simulink library "Linkage_DW_Pullrod_NoSteer"  (R2025a)
settings: Solver=VariableStepAuto  StartTime=0.0  StopTime=10.0  RelTol=1e-3
undefined symbols (not defined in the file): Ac, Af, Ar, InitLinkage, Left, Linkage, Visual, X, Y, Z
libraries: sm_lib x25, Linkage_Arms x5, Suspension_Utilities x4, Linkage_Shock x1, Linkage_Uprights x1
(part 1 of 2)
Description:
  | Component of Simscape Vehicle Templates Library
  | 
  | Copyright 2018-2026 The MathWorks, Inc.
settings Model: Creator=smiller  LastModifiedBy=smiller
settings SolverCC: AlgebraicLoopSolver=TrustRegion
settings DataIOCC: ReturnWorkspaceOutputs=off
settings OptimizationCC: ReuseModelBlockBuffer=off
settings DebuggingCC: UnconnectedInputMsg=warning  UnconnectedOutputMsg=warning  UnconnectedLineMsg=warning  ArithmeticOperatorsInVariantConditions=warning
settings ModelReferenceCC: EnableRefExpFcnMdlSchedulingChecks=on
settings SFSimCC: CustomCodeUndefinedFunction=UseInterfaceOnly
settings RTWCC: GPUComputeCapability=3.5

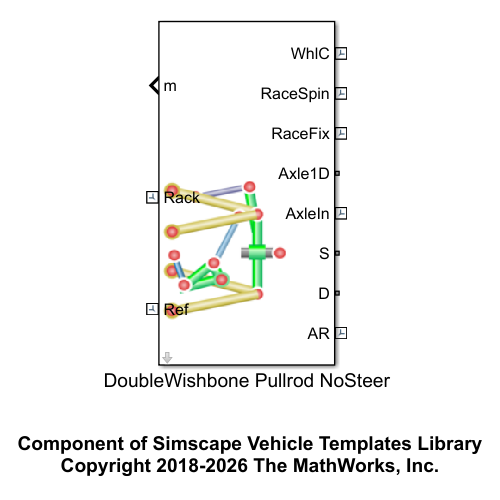
[thumbnail: Simulink's stored preview of the top-level diagram]
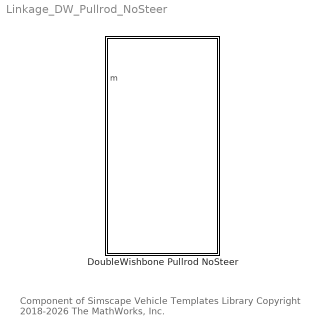
== system Linkage_DW_Pullrod_NoSteer ==
  note: Component of Simscape Vehicle Templates Library
      | Copyright 2018-2026 The MathWorks, Inc.
  DoubleWishbone Pullrod NoSteer : Subsystem  VariantControl=DoubleWishbonePullrodNoSteer  mask(Double-Wishbone Suspension, Pullrod, no Steer){popup_leftRight=Left, hp_in_f_ua=Linkage.UpperWishbone.sInboardF.Value, hp_in_r_ua=Linkage.UpperWishbone.sInboardR.Value, hp_out_ua=Linkage.UpperWishbone.sOutboard.Value, hp_in_f_la=Linkage.LowerWishbone.sInboardF.Value, hp_in_r_la=Linkage.LowerWishbone.sInboardR.Value, hp_out_la=Linkage.LowerWishbone.sOutboard.Value, hp_pullrod_out=Linkage.Pullrod.sUpperArm.Value, hp_pullrod_in=Linkage.Pullrod.sBellcrank.Value, hp_bcr_pivot=Linkage.Bellcrank.sPivot.Value, hp_arb=Linkage.Bellcrank.sAntiRollBar.Value, hp_upr_cg=Linkage.Upright.sCG.Value, hp_upr_wc=Linkage.Upright.sWheelCentre.Value, hp_upr_rod=Linkage.TrackRod.sOutboard.Value, hp_uar_rod=Linkage.TrackRod.sInboard.Value, hp_spr_body=Linkage.Shock.sTop.Value, hp_spr_bcr=Linkage.Shock.sBottom.Value, clr_hp=Visual.hp.clr, opc_hp=Visual.hp.opc, size_hp=Visual.hp.rad, Upper_Arm_to_Subframe=Linkage.Upper_Arm_to_Subframe, ua_mass=Linkage.UpperWishbone.m.Value, clr_ua=Visual.UpperArm.clr, opc_ua=Visual.part.opc, radius_ua=Visual.UpperArm.rad, Lower_Arm_to_Subframe=Linkage.Lower_Arm_to_Subframe, la_mass=Linkage.LowerWishbone.m.Value, clr_la=Visual.LowerArm.clr, opc_la=Visual.part.opc, radius_la=Visual.LowerArm.rad, shock_pist_mass=Linkage.Shock.mPiston.Value, shock_cyl_mass=Linkage.Shock.mCylinder.Value, up_lim_bumpstop=Linkage.Endstop.xMax.Value, low_lim_bumpstop=Linkage.Endstop.xMin.Value, clr_conn_shock=Visual.hp.clr, opc_conn_shock=Visual.hp.opc, size_conn_shock=Visual.hp.rad, clr_shock_cyl=Visual.Shock.cyl.clr, opc_shock_cyl=Visual.part.opc, radius_shock_cyl=Visual.Shock.cyl.rad, clr_shock_piston=Visual.Shock.piston.clr, opc_shock_piston=Visual.part.opc, clr_shock_bumpstop=Visual.Shock.bumpstop.clr, opc_shock_bumpstop=Visual.part.opc, deadvol_len_shock_cyl=Visual.Shock.dead_length, piston_len_shock=Visual.Shock.piston.len, cyl_cap_len_shock=Visual.Shock.cap.len, bumpstop_len_shock=Visual.Shock.bumpstop.len, upr_mass=Linkage.Upright.m.Value, atoe=Linkage.Upright.aToe.Value, acamber=Linkage.Upright.aCamber.Value, axle_len=Linkage.Upright.xAxle.Value, axle_whlc_to_bearing=Linkage.Upright.xWCtoBearing.Value, axle_mass=Linkage.Upright.mAxle.Value, clr_conn_upr=Visual.hp.clr, opc_conn_upr=Visual.hp.opc, size_conn_upr=Visual.hp.rad, clr_upr=Visual.Upright.clr, opc_upr=Visual.part.opc, radius_upr=Visual.Upright.rad, clr_axle=Visual.Axle.clr, opc_axle=Visual.part.opc, radius_axle=Visual.Axle.rad, rod_mass=Linkage.TrackRod.m.Value, clr_conn_rod=Visual.hp.clr, opc_conn_rod=Visual.hp.opc, size_conn_rod=Visual.hp.rad, clr_rod=Visual.TrackRod.clr, opc_rod=Visual.part.opc, radius_rod=Visual.TrackRod.rad, bcr_mass=Linkage.Bellcrank.m.Value, clr_bcr=Visual.Bellcrank.clr, opc_bcr=Visual.part.opc, radius_bcr=Visual.Bellcrank.rad, pullrod_mass=Linkage.Pullrod.m.Value, clr_conn_pullrod=Visual.hp.clr, opc_conn_pullrod=Visual.hp.opc, size_conn_pullrod=Visual.hp.rad, clr_pullrod=Visual.Pullrod.clr, opc_pullrod=Visual.part.opc, radius_pullrod=Visual.Pullrod.rad, whl_init_spd_lr=InitLinkage.nWheel.Value}
      mask prompts: popup_leftRight "Left/Right"; hp_in_f_ua "Upper Arm Front [xyz] (m)"; hp_in_r_ua "Upper Arm Rear [xyz] (m)"; hp_out_ua "Upper Arm Outboard [xyz] (m)"; hp_in_f_la "Lower Arm Front [xyz] (m)"; hp_in_r_la "Lower Arm Rear [xyz] (m)"; hp_out_la "Lower Arm Outboard [xyz] (m)"; hp_pullrod_out "Pullrod Upper Arm [xyz] (m)"; hp_pullrod_in "Pullrod Bellcrank [xyz] (m)"; hp_bcr_pivot "Bellcrank Pivot [xyz] (m)"; hp_arb "HP Bellcrank ARB [xyz] (m)"; hp_upr_cg "Upright CG [xyz] (m)"; hp_upr_wc "Wheel Center [xyz] (m)"; hp_upr_rod "Track Rod Outboard [xyz] (m)"; hp_uar_rod "Track Rod Inboard [xyz] (m)"; hp_spr_body "Spring Body [xyz] (m)"; hp_spr_bcr "Spring Bellcrank [xyz] (m)"; Upper_Arm_to_Subframe "Subframe Connection"; ua_mass "Mass (kg)"; clr_ua "Color [RGB]"; opc_ua "Opacity (0-1)"; radius_ua "Radius (m)"; Lower_Arm_to_Subframe "Subframe Connection"; la_mass "Mass (kg)"; clr_la "Color [RGB]"; opc_la "Opacity (0-1)"; radius_la "Radius (m)"; shock_pist_mass "Piston Mass (kg)"; shock_cyl_mass "Cylinder Mass (kg)"; up_lim_bumpstop "Upper Limit (m)"; low_lim_bumpstop "Lower Limit (m)"; deadvol_len_shock_cyl "Dead Volume Height (m)"; piston_len_shock "Piston Length (m)"; cyl_cap_len_shock "Cylinder Cap Length (m)"; bumpstop_len_shock "Bumpstop Length (m)"; upr_mass "Mass (kg)"; atoe "Toe Angle (deg)"; acamber "Camber Angle (deg)"; axle_len "Axle Length (m)"; axle_whlc_to_bearing "Distance Wheel Ctr to Bearing (m)"; axle_mass "Axle Mass (kg)"; rod_mass "Mass (kg)"; bcr_mass "Mass (kg)"; pullrod_mass "Mass (kg)"; whl_init_spd_lr "Initial Wheel Speed (rad/s)"
      mask help: This models a non-steerable double-wishbone suspension with a rod connecting the upper arm and a bellcrank.
      mask init:
      | if(popup_leftRight == 1)
      |     rhs_susp = 1;
      |     %whlind = 1;
      |     whl_init_spd = whl_init_spd_lr(1);
      | elseif(popup_leftRight == 2)
      |     rhs_susp = -1;
      |     %whlind = 2;
      |     whl_init_spd = whl_init_spd_lr(2);
      | end
      mask Help: web('sm_car_doc_susp_double_wishbone.html')
      mask TypeOptions popup_leftRight:
      | Bellcrank/popup_leftRight | HP Bellcrank/popup_leftRight | HP LA/popup_leftRight | HP UA/popup_leftRight | Hardpoints/popup_leftRight | Lower Arm/popup_leftRight | Pull
      | Rod/popup_leftRight | Track Rod/popup_leftRight | Upper Arm/popup_leftRight | Upright/popup_leftRight
      mask TypeOptions hp_in_f_ua: HP UA/hp_f | Hardpoints/hp_in_f_ua | Upper Arm/hp_in_f
      mask TypeOptions hp_in_r_ua: HP UA/hp_r | Hardpoints/hp_in_r_ua | Upper Arm/hp_in_r
      mask TypeOptions hp_out_ua: Upper Arm/hp_out | Upright/hp_ua_out
      mask TypeOptions hp_in_f_la: HP LA/hp_f | Hardpoints/hp_in_f_la | Lower Arm/hp_in_f
      mask TypeOptions hp_in_r_la: HP LA/hp_r | Hardpoints/hp_in_r_la | Lower Arm/hp_in_r
      mask TypeOptions hp_out_la: Lower Arm/hp_out | Upright/hp_la_out
      mask TypeOptions hp_pullrod_out:
      | Pull
      | Rod/hp_out | Upper Arm/hp_rod
      mask TypeOptions hp_pullrod_in:
      | Bellcrank/hp_rod | HP Bellcrank/hp_2 | Pull
      | Rod/hp_in
      mask TypeOptions hp_bcr_pivot: Bellcrank/hp_bcr_pivot | HP Bellcrank/hp_1 | Hardpoints/hp_bellcrank
      mask TypeOptions hp_arb: Bellcrank/hp_arb
      mask TypeOptions hp_upr_cg: Upright/hp_upr_cg
      mask TypeOptions hp_upr_wc: Upright/hp_upr_wc
      mask TypeOptions hp_upr_rod: Track Rod/hp_out | Upright/hp_upr_rod
      mask TypeOptions hp_uar_rod: Upper Arm/hp_r_upr | Track Rod/hp_in
      mask TypeOptions hp_spr_body: Hardpoints/hp_spr_top | Shock/hp_spr_top
      mask TypeOptions hp_spr_bcr: Bellcrank/hp_bcr_shock | HP Bellcrank/hp_3 | Shock/hp_spr_bot
      mask TypeOptions clr_hp: Hardpoints/clr_hp
      mask TypeOptions opc_hp: Hardpoints/opc_hp
      mask TypeOptions size_hp: Hardpoints/size_hp
      mask TypeOptions ua_mass: Upper Arm/ua_mass
      mask TypeOptions clr_ua: Upper Arm/clr_ua
      mask TypeOptions opc_ua: Upper Arm/opc_ua
      mask TypeOptions radius_ua: Upper Arm/radius_ua
      mask TypeOptions la_mass: Lower Arm/arm_mass
      mask TypeOptions clr_la: Lower Arm/clr_arm
      mask TypeOptions opc_la: Lower Arm/opc_arm
      mask TypeOptions radius_la: Lower Arm/radius_arm
      mask TypeOptions shock_pist_mass: Shock/shock_pist_mass
      mask TypeOptions shock_cyl_mass: Shock/shock_cyl_mass
      mask TypeOptions up_lim_bumpstop: Shock/up_lim_bumpstop
      mask TypeOptions low_lim_bumpstop: Shock/low_lim_bumpstop
      mask TypeOptions clr_conn_shock: Shock/clr_conn_shock
      mask TypeOptions opc_conn_shock: Shock/opc_conn_shock
      mask TypeOptions size_conn_shock: Shock/size_conn_shock
      mask TypeOptions clr_shock_cyl: Shock/clr_shock_cyl
      mask TypeOptions opc_shock_cyl: Shock/opc_shock_cyl
      mask TypeOptions radius_shock_cyl: Shock/radius_shock_cyl
      mask TypeOptions clr_shock_piston: Shock/clr_shock_piston
      mask TypeOptions opc_shock_piston: Shock/opc_shock_piston
      mask TypeOptions clr_shock_bumpstop: Shock/clr_shock_bumpstop
      mask TypeOptions opc_shock_bumpstop: Shock/opc_shock_bumpstop
      mask TypeOptions deadvol_len_shock_cyl: Shock/deadvol_len_shock_cyl
      mask TypeOptions piston_len_shock: Shock/piston_len_shock
      mask TypeOptions cyl_cap_len_shock: Shock/cyl_cap_len_shock
      mask TypeOptions bumpstop_len_shock: Shock/bumpstop_len_shock
      mask TypeOptions upr_mass: Upright/upr_mass
      mask TypeOptions atoe: Upright/atoe
      mask TypeOptions acamber: Upright/acamber
      mask TypeOptions axle_len: Upright/axle_len
      mask TypeOptions axle_whlc_to_bearing: Upright/axle_whlc_to_bearing
      mask TypeOptions axle_mass: Upright/axle_mass
      mask TypeOptions clr_conn_upr: Upright/clr_conn_upr
      mask TypeOptions opc_conn_upr: Upright/opc_conn_upr
      mask TypeOptions size_conn_upr: Upright/size_conn_upr
      mask TypeOptions clr_upr: Upright/clr_upr
      mask TypeOptions opc_upr: Upright/opc_upr
      mask TypeOptions radius_upr: Upright/radius_upr
      mask TypeOptions clr_axle: Upright/clr_axle
      mask TypeOptions opc_axle: Upright/opc_axle
      mask TypeOptions radius_axle: Upright/radius_axle
      mask TypeOptions rod_mass: Track Rod/rod_mass
      mask TypeOptions clr_conn_rod: Track Rod/clr_conn_rod
      mask TypeOptions opc_conn_rod: Track Rod/opc_conn_rod
      mask TypeOptions size_conn_rod: Track Rod/size_conn_rod
      mask TypeOptions clr_rod: Track Rod/clr_rod
      mask TypeOptions opc_rod: Track Rod/opc_rod
      mask TypeOptions radius_rod: Track Rod/radius_rod
      mask TypeOptions bcr_mass: Bellcrank/bcr_mass
      mask TypeOptions clr_bcr: Bellcrank/clr_bcr
      mask TypeOptions opc_bcr: Bellcrank/opc_bcr
      mask TypeOptions radius_bcr: Bellcrank/radius_bcr
      mask TypeOptions pullrod_mass:
      | Pull
      | Rod/rod_mass
      mask TypeOptions clr_conn_pullrod:
      | Pull
      | Rod/clr_conn_rod
      mask TypeOptions opc_conn_pullrod:
      | Pull
      | Rod/opc_conn_rod
      mask TypeOptions size_conn_pullrod:
      | Pull
      | Rod/size_conn_rod
      mask TypeOptions clr_pullrod:
      | Pull
      | Rod/clr_rod
      mask TypeOptions opc_pullrod:
      | Pull
      | Rod/opc_rod
      mask TypeOptions radius_pullrod:
      | Pull
      | Rod/radius_rod
      mask DialogControl cont_hp Prompt: Hardpoints
      mask DialogControl cont_vis_hp Prompt: Visualization
      mask DialogControl text_clr_hp Prompt: Color [RGB]
      mask DialogControl text_opc_hp Prompt: Opac. (0-1)
      mask DialogControl text_size_hp Prompt: Size (m)
      mask DialogControl text_hp Prompt: Hardpoints
      mask DialogControl cont_ua Prompt: UA
      mask DialogControl cont_vis_ua Prompt: Visualization
      mask DialogControl cont_la Prompt: LA
      mask DialogControl cont_vis_la Prompt: Visualization
      mask DialogControl cont_shock Prompt: Shock
      mask DialogControl cont_parts Prompt: Parts
      mask DialogControl cont_bumpstop Prompt: Bumpstop
      mask DialogControl cont_vis_shock Prompt: Visualization
      mask DialogControl text_clr_shock Prompt: Color  [RGB]
      mask DialogControl text_opc_shock Prompt: Opac. (0-1)
      mask DialogControl text_size_shock Prompt: Size (m)
      mask DialogControl text_conn_shock Prompt: Connections
      mask DialogControl text_shock_shock Prompt: Cylinder
      mask DialogControl text_shock_piston Prompt: Piston
      mask DialogControl text_piston_radius Prompt: <cylinder radius>
      mask DialogControl text_shock_bumpstop Prompt: Bumpstop
      mask DialogControl text_bumpstop_radius Prompt: <cylinder radius>
      mask DialogControl cont_upright Prompt: Upright
      mask DialogControl grp_upright Prompt: Upright
      mask DialogControl grp_upright_axle Prompt: Axle
      mask DialogControl cont_vis_upr Prompt: Visualization
      mask DialogControl text_clr_upr Prompt: Color [RGB]
      mask DialogControl text_opc_upr Prompt: Opac. (0-1)
      mask DialogControl text_size_upr Prompt: Size (m)
      mask DialogControl text_conn_upr Prompt: Connections
      mask DialogControl text_upright Prompt: Upright
      mask DialogControl text_axle Prompt: Axle
      mask DialogControl cont_steer Prompt: Steer
      mask DialogControl grp_rod Prompt: Rod
      mask DialogControl cont_vis_rod Prompt: Visualization
      mask DialogControl text_clr_rod Prompt: Color [RGB]
      mask DialogControl text_opc_rod Prompt: Opac. (0-1)
      mask DialogControl text_size_rod Prompt: Size (m)
      mask DialogControl text_conn_rod Prompt: Connections
      mask DialogControl text_rod_rod Prompt: Rod
      mask DialogControl Container23 Prompt: Bellcrank
      mask DialogControl grp_bellcrank Prompt: Bellcrank
      mask DialogControl cont_vis_bellcrank Prompt: Visualization
      mask DialogControl text_clr_bellcrank Prompt: Color [RGB]
      mask DialogControl text_opc_bellcrank Prompt: Opac. (0-1)
      mask DialogControl text_size_bellcrank Prompt: Size (m)
      mask DialogControl text_bellcrank Prompt: Bellcrank
      mask DialogControl cont_pull Prompt: Pullrod
      mask DialogControl grp_pullrod Prompt: Pullrod
      mask DialogControl cont_vis_pullrod Prompt: Visualization
      mask DialogControl text_clr_pullrod Prompt: Color [RGB]
      mask DialogControl text_opc_pullrod Prompt: Opac. (0-1)
      mask DialogControl text_size_pullrod Prompt: Size (m)
      mask DialogControl text_conn_pullrod Prompt: Connections
      mask DialogControl text_pullrod Prompt: Pullrod
      mask DialogControl cont_init Prompt: Initial
      mask Display: image('sm_car_vehicle_linkage_dw_pullrod_noSteer_IMAGE.png');

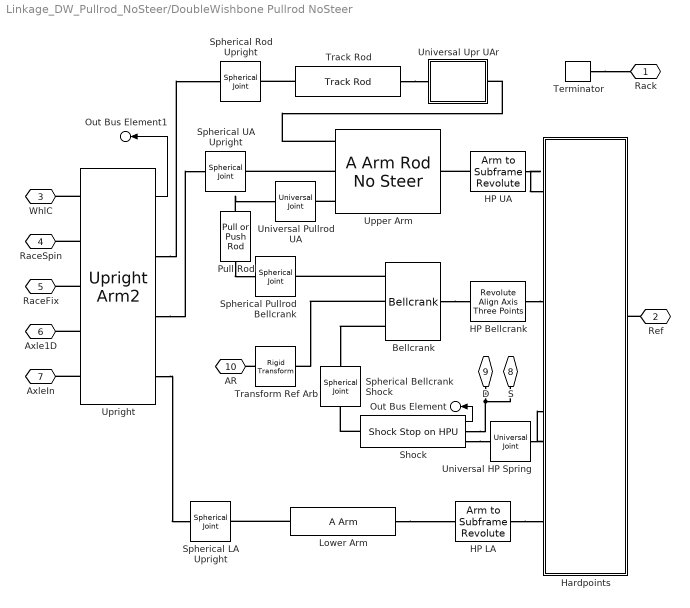
== system Linkage_DW_Pullrod_NoSteer/DoubleWishbone Pullrod NoSteer ==
  Bellcrank : Linkage_Arms/Bellcrank  popup_leftRight=Left  hp_bcr_pivot=hp_bcr_pivot  hp_bcr_shock=hp_spr_bcr  hp_rod=hp_pullrod_in  hp_arb=hp_arb  bcr_mass=bcr_mass  clr_bcr=clr_bcr  opc_bcr=opc_bcr  radius_bcr=radius_bcr
  HP Bellcrank : Suspension_Utilities/Revolute Align Axis Three Points  popup_leftRight=Left  hp_1=hp_bcr_pivot  hp_2=hp_pullrod_in  hp_3=hp_spr_bcr  positionTargetSpecify=on  PositionTargetValue=0
  HP LA : Suspension_Utilities/Arm to Subframe Revolute  VariantControl=Variant1  LabelModeActiveChoice=Rigid_1Rev  popup_leftRight=Left  hp_f=hp_in_f_la  hp_r=hp_in_r_la  Connection=Lower_Arm_to_Subframe  VariantLabel=Lower_Arm_to_Subframe.class.Value
      settings: AttributesFormatString=%<ActiveVariant>
  HP UA : Suspension_Utilities/Arm to Subframe Revolute  VariantControl=Variant1  LabelModeActiveChoice=Rigid_1Rev  popup_leftRight=Left  hp_f=hp_in_f_ua  hp_r=hp_in_r_ua  Connection=Upper_Arm_to_Subframe  VariantLabel=Upper_Arm_to_Subframe.class.Value
      settings: AttributesFormatString=%<ActiveVariant>
  Hardpoints : Subsystem  mask{popup_leftRight=Left, hp_in_f_ua=hp_in_f_ua, hp_in_r_ua=hp_in_r_ua, hp_in_f_la=hp_in_f_la, hp_in_r_la=hp_in_r_la, hp_bellcrank=hp_bcr_pivot, hp_spr_top=hp_spr_body, clr_hp=clr_hp, opc_hp=opc_hp, size_hp=size_hp}
      mask prompts: popup_leftRight "Left/Right"; hp_in_f_ua "Upper Arm Front [xyz] (m)"; hp_in_r_ua "Upper Arm Rear [xyz] (m)"; hp_in_f_la "Lower Arm Front [xyz] (m)"; hp_in_r_la "Lower Arm Rear [xyz] (m)"; hp_bellcrank "Bellcrank Pivot [xyz] (m)"; hp_spr_top "Spring [xyz] (m)"
      mask init:
      | % Set parameter for mirroring (+y or -y)
      | if(popup_leftRight == 1)
      |     rhs_susp = 1;    
      | elseif(popup_leftRight == 2)
      |     rhs_susp = -1;
      | end
      | 
      | rhs_hp = [1 rhs_susp 1];
      mask TypeOptions popup_leftRight: Left | Right
      mask TypeOptions clr_hp: Subsystem/Vis HP LAf/GraphicDiffuseColor | Vis HP LAr/GraphicDiffuseColor | Vis HP Spring/GraphicDiffuseColor | Vis HP UAf/GraphicDiffuseColor | Vis HP UAr/GraphicDiffuseColor
      mask TypeOptions opc_hp: Subsystem/Vis HP LAf/GraphicOpacity | Vis HP LAr/GraphicOpacity | Vis HP Spring/GraphicOpacity | Vis HP UAf/GraphicOpacity | Vis HP UAr/GraphicOpacity
      mask DialogControl cont_hp Prompt: Hardpoints
      mask DialogControl cont_vis_hp Prompt: Visualization
      mask DialogControl text_clr_hp Prompt: Color [RGB]
      mask DialogControl text_opc_hp Prompt: Opac. (0-1)
      mask DialogControl text_size_hp Prompt: Size (m)
      mask DialogControl text_hp Prompt: Hardpoints
      mask Display: image('sm_car_vehicle_linkage_dw_pullrod_hp_IMAGE.png');
  Lower Arm : Linkage_Arms/A Arm  popup_leftRight=Left  hp_in_f=hp_in_f_la  hp_in_r=hp_in_r_la  hp_out=hp_out_la  arm_mass=la_mass  clr_arm=clr_la  opc_arm=opc_la  radius_arm=radius_la
  Pull Rod : Linkage_Arms/Pull or Push Rod  VariantControl=Steer  popup_leftRight=Left  hp_in=hp_pullrod_in  hp_out=hp_pullrod_out  rod_mass=pullrod_mass  clr_conn_rod=clr_conn_pullrod  opc_conn_rod=opc_conn_pullrod  size_conn_rod=size_conn_pullrod  clr_rod=clr_pullrod  opc_rod=opc_pullrod  radius_rod=radius_pullrod
  Shock : Linkage_Shock/Shock Stop on HPU  shock_pist_mass=shock_pist_mass  shock_cyl_mass=shock_cyl_mass  hp_spr_top=hp_spr_body  hp_spr_bot=hp_spr_bcr  up_lim_bumpstop=up_lim_bumpstop  low_lim_bumpstop=low_lim_bumpstop  clr_conn_shock=clr_conn_shock  opc_conn_shock=opc_conn_shock  size_conn_shock=size_conn_shock  clr_shock_cyl=clr_shock_cyl  opc_shock_cyl=opc_shock_cyl  radius_shock_cyl=radius_shock_cyl  clr_shock_piston=clr_shock_piston  opc_shock_piston=opc_shock_piston  clr_shock_bumpstop=clr_shock_bumpstop  opc_shock_bumpstop=opc_shock_bumpstop  deadvol_len_shock_cyl=deadvol_len_shock_cyl  piston_len_shock=piston_len_shock  cyl_cap_len_shock=cyl_cap_len_shock  bumpstop_len_shock=bumpstop_len_shock
  Spherical Bellcrank Shock : sm_lib/Joints/Spherical Joint  JointMode=Normal  CompositeWrenchDir=FollowerOnBase  CompositeWrenchFrame=BaseFrame  SenseConstraintForce=off  SenseConstraintTorque=off  SenseTotalForce=off  SenseTotalTorque=off  PositionTargetSpecify=off  PositionTargetPriority=High  PositionTargetRotationMethod=None  PositionTargetFollAlignAxisA=+X  PositionTargetBaseAlignAxisA=+Y  PositionTargetFollAlignAxisB=+Y  PositionTargetBaseAlignAxisB=+Z  PositionTargetRotationStandardAxis=+Z  PositionTargetRotationAngle=0.0  PositionTargetRotationAngleUnits=deg  PositionTargetRotationArbitraryAxis=[0 0 1]  PositionTargetRotationSequenceAxes=FollowerAxes  PositionTargetRotationSequence=XYX  PositionTargetRotationSequenceAngles=[0 0 0]  PositionTargetRotationSequenceAnglesUnits=deg  PositionTargetRotationMatrix=[1 0 0; 0 1 0; 0 0 1]  PositionTargetQuaternion=[1 0 0 0]  VelocityTargetSpecify=off  VelocityTargetPriority=High  VelocityTargetValue=[0 0 0]  VelocityTargetValueUnits=deg/s  VelocityTargetInFollowerFrame=on  EqPosRotationMethod=None  EqPosFollAlignAxisA=+X  EqPosBaseAlignAxisA=+Y  EqPosFollAlignAxisB=+Y  EqPosBaseAlignAxisB=+Z  EqPosRotationStandardAxis=+Z  EqPosRotationAngle=0.0  EqPosRotationAngleUnits=deg  EqPosRotationArbitraryAxis=[0 0 1]  EqPosRotationSequenceAxes=FollowerAxes  EqPosRotationSequence=XYX  EqPosRotationSequenceAngles=[0 0 0]  EqPosRotationSequenceAnglesUnits=deg  EqPosRotationMatrix=[1 0 0; 0 1 0; 0 0 1]  EqPosQuaternion=[1 0 0 0]  SpringStiffness=0  SpringStiffnessUnits=N*m/deg  DampingCoefficient=0  DampingCoefficientUnits=N*m/(deg/s)  LowerLimitSpecify=off  LowerLimitBound=15  LowerLimitBoundUnits=deg  LowerLimitStiffness=1e4  LowerLimitStiffnessUnits=N*m/deg  LowerLimitDamping=10  LowerLimitDampingUnits=N*m/(deg/s)  LowerLimitTransitionRegionWidth=0.1  LowerLimitTransitionRegionWidthUnits=deg  UpperLimitSpecify=off  UpperLimitBound=45  UpperLimitBoundUnits=deg  UpperLimitStiffness=1e4  UpperLimitStiffnessUnits=N*m/deg  UpperLimitDamping=10  UpperLimitDampingUnits=N*m/(deg/s)  UpperLimitTransitionRegionWidth=0.1  UpperLimitTransitionRegionWidthUnits=deg  TorqueActuationMode=NoTorque  ActuateTorqueX=off  ActuateTorqueY=off  ActuateTorqueZ=off  ActuateTorque=off  ActuationFrame=BaseFrame  SensePosition=off  SenseVelocityX=off  SenseVelocityY=off  SenseVelocityZ=off  SenseVelocity=off  SenseAccelerationX=off  SenseAccelerationY=off  SenseAccelerationZ=off  SenseAcceleration=off  SenseLowerLimitTorqueMag=off  SenseUpperLimitTorqueMag=off  SensingFrame=BaseFrame
  Spherical LA Upright : sm_lib/Joints/Spherical Joint  JointMode=Normal  CompositeWrenchDir=FollowerOnBase  CompositeWrenchFrame=BaseFrame  SenseConstraintForce=off  SenseConstraintTorque=off  SenseTotalForce=off  SenseTotalTorque=off  PositionTargetSpecify=off  PositionTargetPriority=Low  PositionTargetRotationMethod=None  PositionTargetFollAlignAxisA=+X  PositionTargetBaseAlignAxisA=+Y  PositionTargetFollAlignAxisB=+Y  PositionTargetBaseAlignAxisB=+Z  PositionTargetRotationStandardAxis=+Z  PositionTargetRotationAngle=0.0  PositionTargetRotationAngleUnits=deg  PositionTargetRotationArbitraryAxis=[0 0 1]  PositionTargetRotationSequenceAxes=FollowerAxes  PositionTargetRotationSequence=XYX  PositionTargetRotationSequenceAngles=[0 0 0]  PositionTargetRotationSequenceAnglesUnits=deg  PositionTargetRotationMatrix=[1 0 0; 0 1 0; 0 0 1]  PositionTargetQuaternion=[1 0 0 0]  VelocityTargetSpecify=off  VelocityTargetPriority=High  VelocityTargetValue=[0 0 0]  VelocityTargetValueUnits=deg/s  VelocityTargetInFollowerFrame=on  EqPosRotationMethod=None  EqPosFollAlignAxisA=+X  EqPosBaseAlignAxisA=+Y  EqPosFollAlignAxisB=+Y  EqPosBaseAlignAxisB=+Z  EqPosRotationStandardAxis=+Z  EqPosRotationAngle=0.0  EqPosRotationAngleUnits=deg  EqPosRotationArbitraryAxis=[0 0 1]  EqPosRotationSequenceAxes=FollowerAxes  EqPosRotationSequence=XYX  EqPosRotationSequenceAngles=[0 0 0]  EqPosRotationSequenceAnglesUnits=deg  EqPosRotationMatrix=[1 0 0; 0 1 0; 0 0 1]  EqPosQuaternion=[1 0 0 0]  SpringStiffness=0  SpringStiffnessUnits=N*m/deg  DampingCoefficient=0  DampingCoefficientUnits=N*m/(deg/s)  LowerLimitSpecify=off  LowerLimitBound=15  LowerLimitBoundUnits=deg  LowerLimitStiffness=1e4  LowerLimitStiffnessUnits=N*m/deg  LowerLimitDamping=10  LowerLimitDampingUnits=N*m/(deg/s)  LowerLimitTransitionRegionWidth=0.1  LowerLimitTransitionRegionWidthUnits=deg  UpperLimitSpecify=off  UpperLimitBound=45  UpperLimitBoundUnits=deg  UpperLimitStiffness=1e4  UpperLimitStiffnessUnits=N*m/deg  UpperLimitDamping=10  UpperLimitDampingUnits=N*m/(deg/s)  UpperLimitTransitionRegionWidth=0.1  UpperLimitTransitionRegionWidthUnits=deg  TorqueActuationMode=NoTorque  ActuateTorqueX=off  ActuateTorqueY=off  ActuateTorqueZ=off  ActuateTorque=off  ActuationFrame=BaseFrame  SensePosition=off  SenseVelocityX=off  SenseVelocityY=off  SenseVelocityZ=off  SenseVelocity=off  SenseAccelerationX=off  SenseAccelerationY=off  SenseAccelerationZ=off  SenseAcceleration=off  SenseLowerLimitTorqueMag=off  SenseUpperLimitTorqueMag=off  SensingFrame=BaseFrame
  Spherical Pullrod Bellcrank : sm_lib/Joints/Spherical Joint  JointMode=Normal  CompositeWrenchDir=FollowerOnBase  CompositeWrenchFrame=BaseFrame  SenseConstraintForce=off  SenseConstraintTorque=off  SenseTotalForce=off  SenseTotalTorque=off  PositionTargetSpecify=off  PositionTargetPriority=High  PositionTargetRotationMethod=None  PositionTargetFollAlignAxisA=+X  PositionTargetBaseAlignAxisA=+Y  PositionTargetFollAlignAxisB=+Y  PositionTargetBaseAlignAxisB=+Z  PositionTargetRotationStandardAxis=+Z  PositionTargetRotationAngle=0.0  PositionTargetRotationAngleUnits=deg  PositionTargetRotationArbitraryAxis=[0 0 1]  PositionTargetRotationSequenceAxes=FollowerAxes  PositionTargetRotationSequence=XYX  PositionTargetRotationSequenceAngles=[0 0 0]  PositionTargetRotationSequenceAnglesUnits=deg  PositionTargetRotationMatrix=[1 0 0; 0 1 0; 0 0 1]  PositionTargetQuaternion=[1 0 0 0]  VelocityTargetSpecify=off  VelocityTargetPriority=High  VelocityTargetValue=[0 0 0]  VelocityTargetValueUnits=deg/s  VelocityTargetInFollowerFrame=on  EqPosRotationMethod=None  EqPosFollAlignAxisA=+X  EqPosBaseAlignAxisA=+Y  EqPosFollAlignAxisB=+Y  EqPosBaseAlignAxisB=+Z  EqPosRotationStandardAxis=+Z  EqPosRotationAngle=0.0  EqPosRotationAngleUnits=deg  EqPosRotationArbitraryAxis=[0 0 1]  EqPosRotationSequenceAxes=FollowerAxes  EqPosRotationSequence=XYX  EqPosRotationSequenceAngles=[0 0 0]  EqPosRotationSequenceAnglesUnits=deg  EqPosRotationMatrix=[1 0 0; 0 1 0; 0 0 1]  EqPosQuaternion=[1 0 0 0]  SpringStiffness=0  SpringStiffnessUnits=N*m/deg  DampingCoefficient=0  DampingCoefficientUnits=N*m/(deg/s)  LowerLimitSpecify=off  LowerLimitBound=15  LowerLimitBoundUnits=deg  LowerLimitStiffness=1e4  LowerLimitStiffnessUnits=N*m/deg  LowerLimitDamping=10  LowerLimitDampingUnits=N*m/(deg/s)  LowerLimitTransitionRegionWidth=0.1  LowerLimitTransitionRegionWidthUnits=deg  UpperLimitSpecify=off  UpperLimitBound=45  UpperLimitBoundUnits=deg  UpperLimitStiffness=1e4  UpperLimitStiffnessUnits=N*m/deg  UpperLimitDamping=10  UpperLimitDampingUnits=N*m/(deg/s)  UpperLimitTransitionRegionWidth=0.1  UpperLimitTransitionRegionWidthUnits=deg  TorqueActuationMode=NoTorque  ActuateTorqueX=off  ActuateTorqueY=off  ActuateTorqueZ=off  ActuateTorque=off  ActuationFrame=BaseFrame  SensePosition=off  SenseVelocityX=off  SenseVelocityY=off  SenseVelocityZ=off  SenseVelocity=off  SenseAccelerationX=off  SenseAccelerationY=off  SenseAccelerationZ=off  SenseAcceleration=off  SenseLowerLimitTorqueMag=off  SenseUpperLimitTorqueMag=off  SensingFrame=BaseFrame
  Spherical Rod Upright : sm_lib/Joints/Spherical Joint  JointMode=Normal  CompositeWrenchDir=FollowerOnBase  CompositeWrenchFrame=BaseFrame  SenseConstraintForce=off  SenseConstraintTorque=off  SenseTotalForce=off  SenseTotalTorque=off  PositionTargetSpecify=off  PositionTargetPriority=High  PositionTargetRotationMethod=None  PositionTargetFollAlignAxisA=+X  PositionTargetBaseAlignAxisA=+Y  PositionTargetFollAlignAxisB=+Y  PositionTargetBaseAlignAxisB=+Z  PositionTargetRotationStandardAxis=+Z  PositionTargetRotationAngle=0.0  PositionTargetRotationAngleUnits=deg  PositionTargetRotationArbitraryAxis=[0 0 1]  PositionTargetRotationSequenceAxes=FollowerAxes  PositionTargetRotationSequence=XYX  PositionTargetRotationSequenceAngles=[0 0 0]  PositionTargetRotationSequenceAnglesUnits=deg  PositionTargetRotationMatrix=[1 0 0; 0 1 0; 0 0 1]  PositionTargetQuaternion=[1 0 0 0]  VelocityTargetSpecify=off  VelocityTargetPriority=High  VelocityTargetValue=[0 0 0]  VelocityTargetValueUnits=deg/s  VelocityTargetInFollowerFrame=on  EqPosRotationMethod=None  EqPosFollAlignAxisA=+X  EqPosBaseAlignAxisA=+Y  EqPosFollAlignAxisB=+Y  EqPosBaseAlignAxisB=+Z  EqPosRotationStandardAxis=+Z  EqPosRotationAngle=0.0  EqPosRotationAngleUnits=deg  EqPosRotationArbitraryAxis=[0 0 1]  EqPosRotationSequenceAxes=FollowerAxes  EqPosRotationSequence=XYX  EqPosRotationSequenceAngles=[0 0 0]  EqPosRotationSequenceAnglesUnits=deg  EqPosRotationMatrix=[1 0 0; 0 1 0; 0 0 1]  EqPosQuaternion=[1 0 0 0]  SpringStiffness=0  SpringStiffnessUnits=N*m/deg  DampingCoefficient=0  DampingCoefficientUnits=N*m/(deg/s)  LowerLimitSpecify=off  LowerLimitBound=15  LowerLimitBoundUnits=deg  LowerLimitStiffness=1e4  LowerLimitStiffnessUnits=N*m/deg  LowerLimitDamping=10  LowerLimitDampingUnits=N*m/(deg/s)  LowerLimitTransitionRegionWidth=0.1  LowerLimitTransitionRegionWidthUnits=deg  UpperLimitSpecify=off  UpperLimitBound=45  UpperLimitBoundUnits=deg  UpperLimitStiffness=1e4  UpperLimitStiffnessUnits=N*m/deg  UpperLimitDamping=10  UpperLimitDampingUnits=N*m/(deg/s)  UpperLimitTransitionRegionWidth=0.1  UpperLimitTransitionRegionWidthUnits=deg  TorqueActuationMode=NoTorque  ActuateTorqueX=off  ActuateTorqueY=off  ActuateTorqueZ=off  ActuateTorque=off  ActuationFrame=BaseFrame  SensePosition=off  SenseVelocityX=off  SenseVelocityY=off  SenseVelocityZ=off  SenseVelocity=off  SenseAccelerationX=off  SenseAccelerationY=off  SenseAccelerationZ=off  SenseAcceleration=off  SenseLowerLimitTorqueMag=off  SenseUpperLimitTorqueMag=off  SensingFrame=BaseFrame
  Spherical UA Upright : sm_lib/Joints/Spherical Joint  JointMode=Normal  CompositeWrenchDir=FollowerOnBase  CompositeWrenchFrame=BaseFrame  SenseConstraintForce=off  SenseConstraintTorque=off  SenseTotalForce=off  SenseTotalTorque=off  PositionTargetSpecify=on  PositionTargetPriority=Low  PositionTargetRotationMethod=None  PositionTargetFollAlignAxisA=+X  PositionTargetBaseAlignAxisA=+Y  PositionTargetFollAlignAxisB=+Y  PositionTargetBaseAlignAxisB=+Z  PositionTargetRotationStandardAxis=+Z  PositionTargetRotationAngle=0.0  PositionTargetRotationAngleUnits=deg  PositionTargetRotationArbitraryAxis=[0 0 1]  PositionTargetRotationSequenceAxes=FollowerAxes  PositionTargetRotationSequence=XYX  PositionTargetRotationSequenceAngles=[0 0 0]  PositionTargetRotationSequenceAnglesUnits=deg  PositionTargetRotationMatrix=[1 0 0; 0 1 0; 0 0 1]  PositionTargetQuaternion=[1 0 0 0]  VelocityTargetSpecify=off  VelocityTargetPriority=High  VelocityTargetValue=[0 0 0]  VelocityTargetValueUnits=deg/s  VelocityTargetInFollowerFrame=on  EqPosRotationMethod=None  EqPosFollAlignAxisA=+X  EqPosBaseAlignAxisA=+Y  EqPosFollAlignAxisB=+Y  EqPosBaseAlignAxisB=+Z  EqPosRotationStandardAxis=+Z  EqPosRotationAngle=0.0  EqPosRotationAngleUnits=deg  EqPosRotationArbitraryAxis=[0 0 1]  EqPosRotationSequenceAxes=FollowerAxes  EqPosRotationSequence=XYX  EqPosRotationSequenceAngles=[0 0 0]  EqPosRotationSequenceAnglesUnits=deg  EqPosRotationMatrix=[1 0 0; 0 1 0; 0 0 1]  EqPosQuaternion=[1 0 0 0]  SpringStiffness=0  SpringStiffnessUnits=N*m/deg  DampingCoefficient=0  DampingCoefficientUnits=N*m/(deg/s)  LowerLimitSpecify=off  LowerLimitBound=15  LowerLimitBoundUnits=deg  LowerLimitStiffness=1e4  LowerLimitStiffnessUnits=N*m/deg  LowerLimitDamping=10  LowerLimitDampingUnits=N*m/(deg/s)  LowerLimitTransitionRegionWidth=0.1  LowerLimitTransitionRegionWidthUnits=deg  UpperLimitSpecify=off  UpperLimitBound=45  UpperLimitBoundUnits=deg  UpperLimitStiffness=1e4  UpperLimitStiffnessUnits=N*m/deg  UpperLimitDamping=10  UpperLimitDampingUnits=N*m/(deg/s)  UpperLimitTransitionRegionWidth=0.1  UpperLimitTransitionRegionWidthUnits=deg  TorqueActuationMode=NoTorque  ActuateTorqueX=off  ActuateTorqueY=off  ActuateTorqueZ=off  ActuateTorque=off  ActuationFrame=BaseFrame  SensePosition=off  SenseVelocityX=off  SenseVelocityY=off  SenseVelocityZ=off  SenseVelocity=off  SenseAccelerationX=off  SenseAccelerationY=off  SenseAccelerationZ=off  SenseAcceleration=off  SenseLowerLimitTorqueMag=off  SenseUpperLimitTorqueMag=off  SensingFrame=BaseFrame
  Terminator : Suspension_Utilities/Terminator  SystemSampleTime=-1  VariantActivationTime=update diagram  EmptyChoice=off  PassThrough=off  PassThroughVariantControl=(default)  EmptyChoiceVariantControl=(default)  AllowFlexibleInterface=on  Latency=0  AutoFrameSizeCalculation=off
  Track Rod : Linkage_Arms/Track Rod  VariantControl=Steer  popup_leftRight=Left  hp_in=hp_uar_rod  hp_out=hp_upr_rod  rod_mass=rod_mass  clr_conn_rod=clr_conn_rod  opc_conn_rod=opc_conn_rod  size_conn_rod=size_conn_rod  clr_rod=clr_rod  opc_rod=opc_rod  radius_rod=radius_rod
  Transform Ref Arb : sm_lib/Frames and Transforms/Rigid Transform  RotationMethod=None  FollAlignAxisA=+X  BaseAlignAxisA=+Y  FollAlignAxisB=+Y  BaseAlignAxisB=+Z  RotationStandardAxis=+Z  RotationAngle=0.0  RotationAngleUnits=deg  RotationArbitraryAxis=[0 0 1]  RotationSequenceAxes=FollowerAxes  RotationSequence=XYX  RotationSequenceAngles=[0 0 0]  RotationSequenceAnglesUnits=deg  RotationMatrix=[1 0 0; 0 1 0; 0 0 1]  Quaternion=[1 0 0 0]  TranslationMethod=Cartesian  TranslationCartesianOffset=hp_arb.*[1 rhs_susp 1]  TranslationCartesianOffsetUnits=m  TranslationStandardAxis=+Z  TranslationStandardOffset=0  TranslationStandardOffsetUnits=m  TranslationROffset=0  TranslationROffsetUnits=m  TranslationThetaOffset=0  TranslationThetaOffsetUnits=deg  TranslationZOffset=0  TranslationZOffsetUnits=m
  Universal HP Spring : sm_lib/Joints/Universal Joint  JointMode=Normal  CompositeWrenchDir=FollowerOnBase  CompositeWrenchFrame=BaseFrame  SenseConstraintForce=off  SenseConstraintTorque=off  SenseTotalForce=off  SenseTotalTorque=off  RxPositionTargetSpecify=off  RxPositionTargetPriority=High  RxPositionTargetValue=0  RxPositionTargetValueUnits=deg  RxVelocityTargetSpecify=off  RxVelocityTargetPriority=High  RxVelocityTargetValue=0  RxVelocityTargetValueUnits=deg/s  RxEquilibriumPosition=0  RxEquilibriumPositionUnits=deg  RxSpringStiffness=0  RxSpringStiffnessUnits=N*m/deg  RxDampingCoefficient=0  RxDampingCoefficientUnits=N*m/(deg/s)  RxLowerLimitSpecify=off  RxLowerLimitBound=-90  RxLowerLimitBoundUnits=deg  RxLowerLimitStiffness=1e4  RxLowerLimitStiffnessUnits=N*m/deg  RxLowerLimitDamping=10  RxLowerLimitDampingUnits=N*m/(deg/s)  RxLowerLimitTransitionRegionWidth=0.1  RxLowerLimitTransitionRegionWidthUnits=deg  RxUpperLimitSpecify=off  RxUpperLimitBound=90  RxUpperLimitBoundUnits=deg  RxUpperLimitStiffness=1e4  RxUpperLimitStiffnessUnits=N*m/deg  RxUpperLimitDamping=10  RxUpperLimitDampingUnits=N*m/(deg/s)  RxUpperLimitTransitionRegionWidth=0.1  RxUpperLimitTransitionRegionWidthUnits=deg  RxTorqueActuationMode=NoTorque  RxMotionActuationMode=ComputedMotion  RxSensePosition=off  RxSenseVelocity=off  RxSenseAcceleration=off  RxSenseTorqueForce=off  RxSenseLowerLimitTorqueForce=off  RxSenseUpperLimitTorqueForce=off  RyPositionTargetSpecify=off  RyPositionTargetPriority=High  RyPositionTargetValue=0  RyPositionTargetValueUnits=deg  RyVelocityTargetSpecify=off  RyVelocityTargetPriority=High  RyVelocityTargetValue=0  RyVelocityTargetValueUnits=deg/s  RyEquilibriumPosition=0  RyEquilibriumPositionUnits=deg  RySpringStiffness=0  RySpringStiffnessUnits=N*m/deg  RyDampingCoefficient=0  RyDampingCoefficientUnits=N*m/(deg/s)  RyLowerLimitSpecify=off  RyLowerLimitBound=-90  RyLowerLimitBoundUnits=deg  RyLowerLimitStiffness=1e4  RyLowerLimitStiffnessUnits=N*m/deg  RyLowerLimitDamping=10  RyLowerLimitDampingUnits=N*m/(deg/s)  RyLowerLimitTransitionRegionWidth=0.1  RyLowerLimitTransitionRegionWidthUnits=deg  RyUpperLimitSpecify=off  RyUpperLimitBound=90  RyUpperLimitBoundUnits=deg  RyUpperLimitStiffness=1e4  RyUpperLimitStiffnessUnits=N*m/deg  RyUpperLimitDamping=10  RyUpperLimitDampingUnits=N*m/(deg/s)  RyUpperLimitTransitionRegionWidth=0.1  RyUpperLimitTransitionRegionWidthUnits=deg  RyTorqueActuationMode=NoTorque  RyMotionActuationMode=ComputedMotion  RySensePosition=off  RySenseVelocity=off  RySenseAcceleration=off  RySenseTorqueForce=off  RySenseLowerLimitTorqueForce=off  RySenseUpperLimitTorqueForce=off
  Universal Pullrod UA : sm_lib/Joints/Universal Joint  JointMode=Normal  CompositeWrenchDir=FollowerOnBase  CompositeWrenchFrame=BaseFrame  SenseConstraintForce=off  SenseConstraintTorque=off  SenseTotalForce=off  SenseTotalTorque=off  RxPositionTargetSpecify=off  RxPositionTargetPriority=High  RxPositionTargetValue=0  RxPositionTargetValueUnits=deg  RxVelocityTargetSpecify=off  RxVelocityTargetPriority=High  RxVelocityTargetValue=0  RxVelocityTargetValueUnits=deg/s  RxEquilibriumPosition=0  RxEquilibriumPositionUnits=deg  RxSpringStiffness=0  RxSpringStiffnessUnits=N*m/deg  RxDampingCoefficient=0  RxDampingCoefficientUnits=N*m/(deg/s)  RxLowerLimitSpecify=off  RxLowerLimitBound=-90  RxLowerLimitBoundUnits=deg  RxLowerLimitStiffness=1e4  RxLowerLimitStiffnessUnits=N*m/deg  RxLowerLimitDamping=10  RxLowerLimitDampingUnits=N*m/(deg/s)  RxLowerLimitTransitionRegionWidth=0.1  RxLowerLimitTransitionRegionWidthUnits=deg  RxUpperLimitSpecify=off  RxUpperLimitBound=90  RxUpperLimitBoundUnits=deg  RxUpperLimitStiffness=1e4  RxUpperLimitStiffnessUnits=N*m/deg  RxUpperLimitDamping=10  RxUpperLimitDampingUnits=N*m/(deg/s)  RxUpperLimitTransitionRegionWidth=0.1  RxUpperLimitTransitionRegionWidthUnits=deg  RxTorqueActuationMode=NoTorque  RxMotionActuationMode=ComputedMotion  RxSensePosition=off  RxSenseVelocity=off  RxSenseAcceleration=off  RxSenseTorqueForce=off  RxSenseLowerLimitTorqueForce=off  RxSenseUpperLimitTorqueForce=off  RyPositionTargetSpecify=off  RyPositionTargetPriority=High  RyPositionTargetValue=0  RyPositionTargetValueUnits=deg  RyVelocityTargetSpecify=off  RyVelocityTargetPriority=High  RyVelocityTargetValue=0  RyVelocityTargetValueUnits=deg/s  RyEquilibriumPosition=0  RyEquilibriumPositionUnits=deg  RySpringStiffness=0  RySpringStiffnessUnits=N*m/deg  RyDampingCoefficient=0  RyDampingCoefficientUnits=N*m/(deg/s)  RyLowerLimitSpecify=off  RyLowerLimitBound=-90  RyLowerLimitBoundUnits=deg  RyLowerLimitStiffness=1e4  RyLowerLimitStiffnessUnits=N*m/deg  RyLowerLimitDamping=10  RyLowerLimitDampingUnits=N*m/(deg/s)  RyLowerLimitTransitionRegionWidth=0.1  RyLowerLimitTransitionRegionWidthUnits=deg  RyUpperLimitSpecify=off  RyUpperLimitBound=90  RyUpperLimitBoundUnits=deg  RyUpperLimitStiffness=1e4  RyUpperLimitStiffnessUnits=N*m/deg  RyUpperLimitDamping=10  RyUpperLimitDampingUnits=N*m/(deg/s)  RyUpperLimitTransitionRegionWidth=0.1  RyUpperLimitTransitionRegionWidthUnits=deg  RyTorqueActuationMode=NoTorque  RyMotionActuationMode=ComputedMotion  RySensePosition=off  RySenseVelocity=off  RySenseAcceleration=off  RySenseTorqueForce=off  RySenseLowerLimitTorqueForce=off  RySenseUpperLimitTorqueForce=off
  Universal Upr UAr : Subsystem
      mask Display: image('sm_car_variant_universal.png');
  Upper Arm : Linkage_Arms/A Arm Rod No Steer  popup_leftRight=Left  hp_in_f=hp_in_f_ua  hp_in_r=hp_in_r_ua  hp_r_upr=hp_uar_rod  hp_out=hp_out_ua  hp_rod=hp_pullrod_out  ua_mass=ua_mass  clr_solid=clr_ua  opc_solid=opc_ua  rad_solid=radius_ua
  Upright : Linkage_Uprights/Upright Arm2  popup_leftRight=Left  hp_ua_out=hp_out_ua  hp_la_out=hp_out_la  hp_upr_rod=hp_upr_rod  hp_upr_cg=hp_upr_cg  hp_upr_wc=hp_upr_wc  axle_len=axle_len  axle_whlc_to_bearing=axle_whlc_to_bearing  axle_mass=axle_mass  atoe=atoe  acamber=acamber  upr_mass=upr_mass  whl_init_spd_upr=whl_init_spd  clr_conn_upr=clr_conn_upr  opc_conn_upr=opc_conn_upr  size_conn_upr=size_conn_upr  clr_upr=clr_upr  opc_upr=opc_upr  radius_upr=radius_upr  clr_axle=clr_axle  opc_axle=opc_axle  radius_axle=radius_axle
  Rack : PMIOPort  Side=Right
  Ref : PMIOPort  Port=2  Side=Right
  WhlC : PMIOPort  Port=3  Side=Left
  RaceSpin : PMIOPort  Port=4  Side=Left
  RaceFix : PMIOPort  Port=5  Side=Left
  Axle1D : PMIOPort  Port=6  Side=Left
  AxleIn : PMIOPort  Port=7  Side=Left
  S : PMIOPort  Port=8  Side=Left
  D : PMIOPort  Port=9  Side=Left
  AR : PMIOPort  Port=10  Side=Left
  Out Bus Element : Outport  VectorParamsAs1DForOutWhenUnconnected=off  PortName=m  Element=Shock
  Out Bus Element1 : Outport  VectorParamsAs1DForOutWhenUnconnected=off  PortName=m  Element=Upright
  wires:
  Shock/1 -> Out Bus Element/1
  Upright/1 -> Out Bus Element1/1
  connections:
  Bellcrank/LConn3 -- Spherical Bellcrank Shock/LConn1
  Universal HP Spring/LConn1 -- Hardpoints/LConn3
  Shock/LConn1 -- Spherical Bellcrank Shock/RConn1
  HP Bellcrank/LConn1 -- Hardpoints/LConn2
  Pull Rod/RConn1 -- Spherical Pullrod Bellcrank/LConn1
  Bellcrank/LConn1 -- Spherical Pullrod Bellcrank/RConn1
  Pull Rod/LConn1 -- Universal Pullrod UA/LConn1
  Bellcrank/LConn2 -- Transform Ref Arb/RConn1
  Upper Arm/LConn3 -- Universal Pullrod UA/RConn1
  Bellcrank/RConn1 -- HP Bellcrank/RConn1
  Shock/RConn1 -- S/RConn1 -- D/RConn1
  Transform Ref Arb/LConn1 -- AR/RConn1
  Track Rod/RConn1 -- Universal Upr UAr/LConn1
  Track Rod/LConn1 -- Spherical Rod Upright/LConn1
  Upright/RConn2 -- Spherical UA Upright/RConn1
  Lower Arm/LConn1 -- Spherical LA Upright/LConn1
  Lower Arm/RConn1 -- HP LA/RConn1
  Upper Arm/LConn2 -- Spherical UA Upright/LConn1
  Upright/RConn3 -- Spherical LA Upright/RConn1
  HP LA/LConn1 -- Hardpoints/LConn4
  HP UA/RConn1 -- Upper Arm/RConn1
  Upright/LConn4 -- Axle1D/RConn1
  Upright/RConn1 -- Spherical Rod Upright/RConn1
  HP UA/LConn1 -- Hardpoints/LConn1
  Ref/RConn1 -- Hardpoints/RConn1
  Upright/LConn1 -- WhlC/RConn1
  Shock/RConn2 -- Universal HP Spring/RConn1
  Upright/LConn2 -- RaceSpin/RConn1
  Upright/LConn3 -- RaceFix/RConn1
  Upright/LConn5 -- AxleIn/RConn1
  Upper Arm/LConn1 -- Universal Upr UAr/RConn1
  Terminator/RConn1 -- Rack/RConn1
